simulink model "diffdrive_sim"  (R2024a)
settings: Solver=ode4  StartTime=0.0  StopTime=10  FixedStep=0.001  RelTol=1e-3
settings Model: Creator=bai  LastModifiedBy=bai

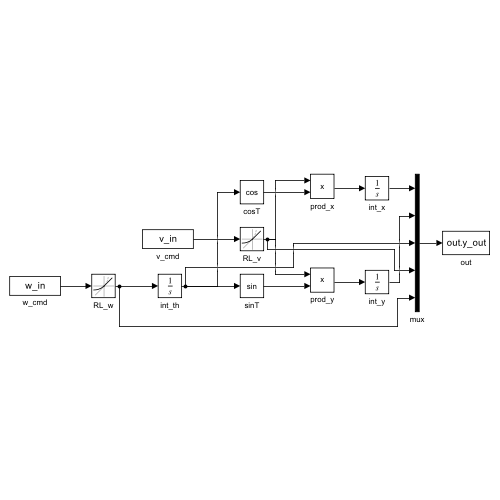
[thumbnail: Simulink's stored preview of the top-level diagram]
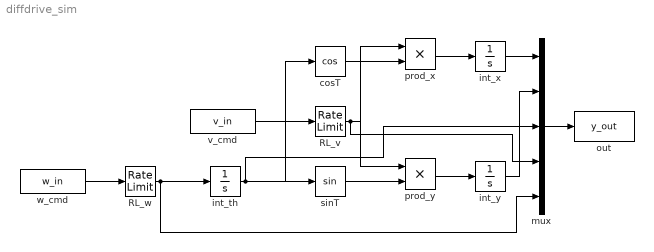
== system diffdrive_sim ==
  RL_v : RateLimiter  RisingSlewLimit=1.0  FallingSlewLimit=-2.0  SampleTimeMode=inherited
  RL_w : RateLimiter  RisingSlewLimit=3.0  FallingSlewLimit=-6.0  SampleTimeMode=inherited
  cosT : Trigonometry  Operator=cos
  int_th : Integrator
  int_x : Integrator
  int_y : Integrator
  mux : Mux  Inputs=5
  out : ToWorkspace  VariableName=y_out  SampleTime=-1
  prod_x : Product
  prod_y : Product
  sinT : Trigonometry
  v_cmd : FromWorkspace  VariableName=v_in  Interpolate=off  OutputAfterFinalValue=Holding final value
  w_cmd : FromWorkspace  VariableName=w_in  Interpolate=off  OutputAfterFinalValue=Holding final value
  wires:
  sinT/1 -> prod_y/2
  int_th/1 -> sinT/1, cosT/1, mux/3
  cosT/1 -> prod_x/2
  w_cmd/1 -> RL_w/1
  RL_w/1 -> int_th/1, mux/5
  v_cmd/1 -> RL_v/1
  RL_v/1 -> mux/4, prod_x/1, prod_y/1
  prod_y/1 -> int_y/1
  prod_x/1 -> int_x/1
  int_x/1 -> mux/1
  int_y/1 -> mux/2
  mux/1 -> out/1
